simulink model "F2026_ECE597_01_Open_Loop_Step_Response"  (R2025a)
settings: Solver=VariableStepAuto  StartTime=0.0  StopTime=10.0  RelTol=1e-3
values from neighbouring files (symbols this model uses):
  A = [[-0.59 0.92 0.61 -9.82]; [-0.23 -6.31 4.42 0.19]; [ 0.78 -5.59 -5.92 0]; [0 0 1 0]]    [F2026_ECE597_01_Open_Loop_Step_Response.m]
  B = [[4.26 19.43 0.59 0.01 -0.92]; [-58.88 0.25 0.23 0.02 6.31]; [-101.91 0 -0.78 0 5.59]; [0 0 0 0 0]]    [F2026_ECE597_01_Open_Loop_Step_Response.m]
  C = eye(4)    [F2026_ECE597_01_Open_Loop_Step_Response.m]
  D = zeros(4, 5)    [F2026_ECE597_01_Open_Loop_Step_Response.m]
settings Model: Creator=gresham2  LastModifiedBy=gresham2

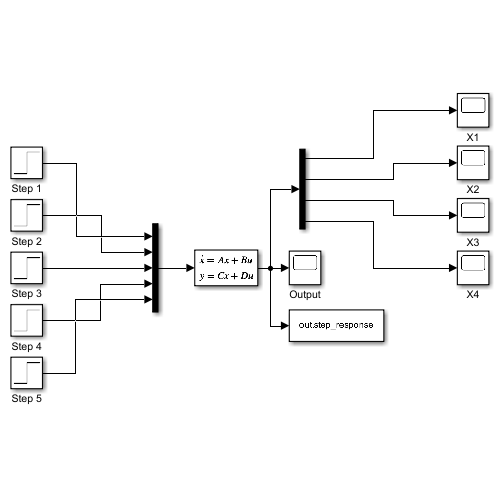
[thumbnail: Simulink's stored preview of the top-level diagram]
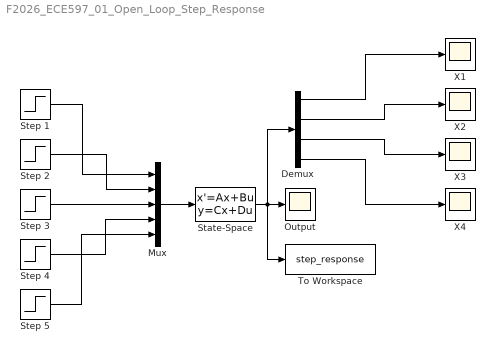
== system F2026_ECE597_01_Open_Loop_Step_Response ==
  Demux : Demux
  Mux : Mux  Inputs=5
  Output : Scope
      settings: ActiveDisplayYMinimum=-6.9431651149116629  ActiveDisplayYMaximum=5.2284333780818315
  State-Space : StateSpace  A=A  B=B  C=C  D=D  InitialCondition=0
  Step {1..5} (5 alike) : Step  SampleTime=0
  To Workspace : ToWorkspace  VariableName=step_response  SaveFormat=Timeseries  SampleTime=-1
  X{1..4} (4 alike) : Scope
      X1 settings: ActiveDisplayYMinimum=-23.407240250375082  ActiveDisplayYMaximum=89.4462657581779
      X2 settings: ActiveDisplayYMinimum=-1  ActiveDisplayYMaximum=1  DataLoggingVariableName=ScopeData2
      X3 settings: ActiveDisplayYMinimum=-1  ActiveDisplayYMaximum=1  DataLoggingVariableName=ScopeData3
      X4 settings: ActiveDisplayYMinimum=-1  ActiveDisplayYMaximum=1  DataLoggingVariableName=ScopeData4
  wires:
  State-Space/1 -> To Workspace/1, Demux/1, Output/1
  Step 3/1 -> Mux/3
  Step 2/1 -> Mux/2
  Step 1/1 -> Mux/1
  Step 4/1 -> Mux/4
  Step 5/1 -> Mux/5
  Mux/1 -> State-Space/1
  Demux/2 -> X2/1
  Demux/3 -> X3/1
  Demux/1 -> X1/1
  Demux/4 -> X4/1
